simulink model "winder_mechanics"  (R2026a)
settings: Solver=VariableStepAuto  StopTime=Tsim  MaxStep=1e-3  RelTol=1e-4
undefined symbols (not defined in the file): draw_max, F_ref, Ki_draw, Ki_speed, Kp_draw, Kp_speed, Tmax, v_init, v_max, v_slope, winder_mode
libraries: slpidlib x2, simulink x1
settings Model: Creator=kunal  LastModifiedBy=kunal

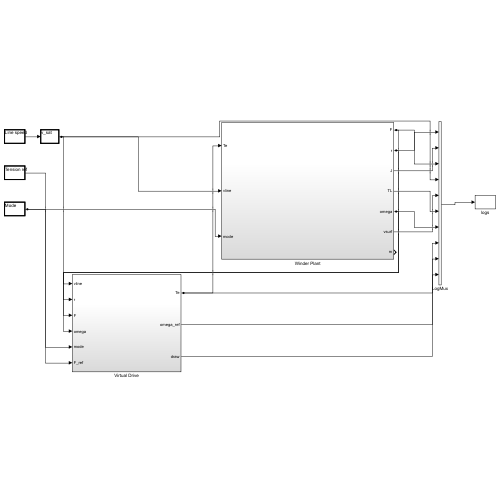
[thumbnail: Simulink's stored preview of the top-level diagram]
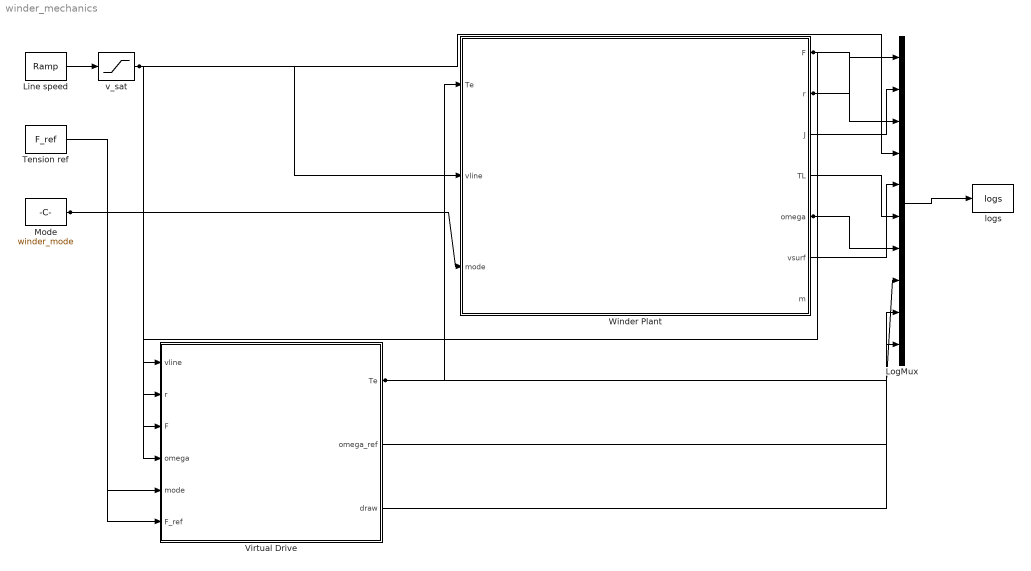
== system winder_mechanics ==
  Line speed : simulink/Sources/Ramp  slope=v_slope  start=0  InitialOutput=v_init
  LogMux : Mux  Inputs=10
  Mode : Constant  Value=winder_mode
  Tension ref : Constant  Value=F_ref
  Virtual Drive : Subsystem
  Winder Plant : Subsystem
  logs : ToWorkspace  VariableName=logs  SaveFormat=Timeseries  SampleTime=-1
  v_sat : Saturate  UpperLimit=v_max  LowerLimit=0
  wires:
  Line speed/1 -> v_sat/1
  v_sat/1 -> Winder Plant/2(vline), Virtual Drive/1(vline), LogMux/4
  Tension ref/1 -> Virtual Drive/6(F_ref)
  Mode/1 -> Winder Plant/3(mode), Virtual Drive/5(mode)
  Winder Plant/2(r) -> Virtual Drive/2(r), LogMux/1
  Winder Plant/1(F) -> Virtual Drive/3(F), LogMux/3
  Winder Plant/5(omega) -> Virtual Drive/4(omega), LogMux/7
  Virtual Drive/1(Te) -> Winder Plant/1(Te), LogMux/8
  Winder Plant/3(J) -> LogMux/2
  Winder Plant/6(vsurf) -> LogMux/5
  Winder Plant/4(TL) -> LogMux/6
  Virtual Drive/2(omega_ref) -> LogMux/9
  Virtual Drive/3(draw) -> LogMux/10
  LogMux/1 -> logs/1

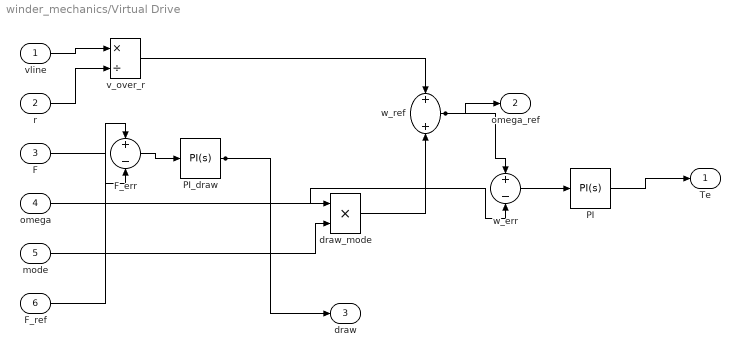
== system winder_mechanics/Virtual Drive ==
  vline : Inport
  r : Inport  Port=2
  F : Inport  Port=3
  omega : Inport  Port=4
  mode : Inport  Port=5
  F_ref : Inport  Port=6
  F_err : Sum  Inputs=+-
  PI : slpidlib/PID Controller  Controller=PI  Form=Parallel  TimeDomain=Continuous-time  UseExternalTs=off  SampleTime=-1  IntegratorMethod=Forward Euler  FilterMethod=Forward Euler  ControllerParametersSource=internal  P=Kp_speed  I=Ki_speed  UseKiTs=off  D=0  UseExternalDerivativeSource=off  N=100  UseFilter=on  TunerSelectOption=Transfer Function Based (PID Tuner App)  InitialConditionSource=internal  InitialConditionForIntegrator=Te0  InitialConditionForFilter=0  DifferentiatorICPrevScaledInput=0  ExternalReset=none  TrackingMode=off  Kt=1  LimitOutput=on  SatLimitsSource=internal  UpperSaturationLimit=Tmax  LowerSaturationLimit=-Tmax  LinearizeAsGain=on  AntiWindupMode=clamping  Kb=1  LimitIntegrator=off  UpperIntegratorSaturationLimit=inf  LowerIntegratorSaturationLimit=-inf  POutMin=[]  POutMax=[]  IOutMin=[]  IOutMax=[]  DOutMin=[]  DOutMax=[]  NOutMin=[]  NOutMax=[]  SumOutMin=[]  SumOutMax=[]  SaturationOutMin=[]  SaturationOutMax=[]  PParamMin=[]  PParamMax=[]  IParamMin=[]  IParamMax=[]  DParamMin=[]  DParamMax=[]  NParamMin=[]  NParamMax=[]  KbParamMin=[]  KbParamMax=[]  KtParamMin=[]  KtParamMax=[]  KbOutMin=[]  KbOutMax=[]  KtOutMin=[]  KtOutMax=[]  IntegratorOutMin=[]  IntegratorOutMax=[]  FilterOutMin=[]  FilterOutMax=[]  SumI1OutMin=[]  SumI1OutMax=[]  SumI2OutMin=[]  SumI2OutMax=[]  SumI3OutMin=[]  SumI3OutMax=[]  SumI4OutMin=[]  SumI4OutMax=[]  SumDOutMin=[]  SumDOutMax=[]  DifferentiatorOutMin=[]  DifferentiatorOutMax=[]  FilterDiffOutCoefMin=[]  FilterDiffOutCoefMax=[]  ReciprocalOutMin=[]  ReciprocalOutMax=[]  SumDenOutMin=[]  SumDenOutMax=[]  SumNumOutMin=[]  SumNumOutMax=[]  DivideOutMin=[]  DivideOutMax=[]  UdiffTsProdOutMin=[]  UdiffTsProdOutMax=[]  NTsProdOutMin=[]  NTsProdOutMax=[]  UintegralTsProdOutMin=[]  UintegralTsProdOutMax=[]  UngainTsProdOutMin=[]  UngainTsProdOutMax=[]  ClampingZeroOutDataTypeStr=Inherit: Inherit via back propagation  ClampingZeroOutMin=[]  ClampingZeroOutMax=[]  FilterDenConstantOutDataTypeStr=Inherit: Inherit via back propagation  FilterDenConstantOutMin=[]  FilterDenConstantOutMax=[]  PCopyOutDataTypeStr=Inherit: Inherit via back propagation  PCopyOutMin=[]  PCopyOutMax=[]  NCopyOutDataTypeStr=Inherit: Inherit via back propagation  NCopyOutMin=[]  NCopyOutMax=[]  IntegratorContinuousStateAttributes=''  IntegratorStateMustResolveToSignalObject=off  IntegratorRTWStateStorageClass=Auto  FilterContinuousStateAttributes=''  FilterStateMustResolveToSignalObject=off  FilterRTWStateStorageClass=Auto  ParallelPVariant=InternalParameters  IdealPVariant=Disabled  IVariant=InternalParameters  DVariant=Disabled  IntegratorVariant=Continuous  SatVariant=Enabled  AWVariant=ContClampingParallel  PCopyVariant=Disabled  TRVariant=Disabled  FdbkBlocksVariant=Forward  IdealPFdbkVariant=Disabled  SatFdbkVariant=Disabled  DerivativeFilterVariant=Disabled  NVariant=Disabled  NCopyVariant=Disabled_SignalSpec  FilterICVariant=Disabled  IntegratorICVariant=InternalICs  ExternalResetVariant=Disabled  TRSumVariant=Passthrough  SumFdbkVariant=Disabled  SumVariant=Sum_PI  TsampFilterVariant=InternalTs  TsampNgainVariant=Passthrough  TsampIntegralVariant=Disabled_SignalSpec  ExternalSaturationOutDataTypeStr=Inherit: Same as second input  DerivativeSourceVariant=Disabled  PreIntVariant=InternalPreInt
  PI_draw : slpidlib/PID Controller  Controller=PI  Form=Parallel  TimeDomain=Continuous-time  UseExternalTs=off  SampleTime=-1  IntegratorMethod=Forward Euler  FilterMethod=Forward Euler  ControllerParametersSource=internal  P=Kp_draw  I=Ki_draw  UseKiTs=off  D=0  UseExternalDerivativeSource=off  N=100  UseFilter=on  TunerSelectOption=Transfer Function Based (PID Tuner App)  InitialConditionSource=internal  InitialConditionForIntegrator=0  InitialConditionForFilter=0  DifferentiatorICPrevScaledInput=0  ExternalReset=none  TrackingMode=off  Kt=1  LimitOutput=on  SatLimitsSource=internal  UpperSaturationLimit=draw_max  LowerSaturationLimit=-draw_max  LinearizeAsGain=on  AntiWindupMode=clamping  Kb=1  LimitIntegrator=off  UpperIntegratorSaturationLimit=inf  LowerIntegratorSaturationLimit=-inf  POutMin=[]  POutMax=[]  IOutMin=[]  IOutMax=[]  DOutMin=[]  DOutMax=[]  NOutMin=[]  NOutMax=[]  SumOutMin=[]  SumOutMax=[]  SaturationOutMin=[]  SaturationOutMax=[]  PParamMin=[]  PParamMax=[]  IParamMin=[]  IParamMax=[]  DParamMin=[]  DParamMax=[]  NParamMin=[]  NParamMax=[]  KbParamMin=[]  KbParamMax=[]  KtParamMin=[]  KtParamMax=[]  KbOutMin=[]  KbOutMax=[]  KtOutMin=[]  KtOutMax=[]  IntegratorOutMin=[]  IntegratorOutMax=[]  FilterOutMin=[]  FilterOutMax=[]  SumI1OutMin=[]  SumI1OutMax=[]  SumI2OutMin=[]  SumI2OutMax=[]  SumI3OutMin=[]  SumI3OutMax=[]  SumI4OutMin=[]  SumI4OutMax=[]  SumDOutMin=[]  SumDOutMax=[]  DifferentiatorOutMin=[]  DifferentiatorOutMax=[]  FilterDiffOutCoefMin=[]  FilterDiffOutCoefMax=[]  ReciprocalOutMin=[]  ReciprocalOutMax=[]  SumDenOutMin=[]  SumDenOutMax=[]  SumNumOutMin=[]  SumNumOutMax=[]  DivideOutMin=[]  DivideOutMax=[]  UdiffTsProdOutMin=[]  UdiffTsProdOutMax=[]  NTsProdOutMin=[]  NTsProdOutMax=[]  UintegralTsProdOutMin=[]  UintegralTsProdOutMax=[]  UngainTsProdOutMin=[]  UngainTsProdOutMax=[]  ClampingZeroOutDataTypeStr=Inherit: Inherit via back propagation  ClampingZeroOutMin=[]  ClampingZeroOutMax=[]  FilterDenConstantOutDataTypeStr=Inherit: Inherit via back propagation  FilterDenConstantOutMin=[]  FilterDenConstantOutMax=[]  PCopyOutDataTypeStr=Inherit: Inherit via back propagation  PCopyOutMin=[]  PCopyOutMax=[]  NCopyOutDataTypeStr=Inherit: Inherit via back propagation  NCopyOutMin=[]  NCopyOutMax=[]  IntegratorContinuousStateAttributes=''  IntegratorStateMustResolveToSignalObject=off  IntegratorRTWStateStorageClass=Auto  FilterContinuousStateAttributes=''  FilterStateMustResolveToSignalObject=off  FilterRTWStateStorageClass=Auto  ParallelPVariant=InternalParameters  IdealPVariant=Disabled  IVariant=InternalParameters  DVariant=Disabled  IntegratorVariant=Continuous  SatVariant=Enabled  AWVariant=ContClampingParallel  PCopyVariant=Disabled  TRVariant=Disabled  FdbkBlocksVariant=Forward  IdealPFdbkVariant=Disabled  SatFdbkVariant=Disabled  DerivativeFilterVariant=Disabled  NVariant=Disabled  NCopyVariant=Disabled_SignalSpec  FilterICVariant=Disabled  IntegratorICVariant=InternalICs  ExternalResetVariant=Disabled  TRSumVariant=Passthrough  SumFdbkVariant=Disabled  SumVariant=Sum_PI  TsampFilterVariant=InternalTs  TsampNgainVariant=Passthrough  TsampIntegralVariant=Disabled_SignalSpec  ExternalSaturationOutDataTypeStr=Inherit: Same as second input  DerivativeSourceVariant=Disabled  PreIntVariant=InternalPreInt
  draw_mode : Product
  v_over_r : Product  Inputs=*/
  w_err : Sum  Inputs=+-
  w_ref : Sum
  Te : Outport
  omega_ref : Outport  Port=2
  draw : Outport  Port=3
  wires:
  vline/1 -> v_over_r/1
  r/1 -> v_over_r/2
  F_ref/1 -> F_err/1
  F/1 -> F_err/2
  F_err/1 -> PI_draw/1
  PI_draw/1 -> draw_mode/1, draw/1
  mode/1 -> draw_mode/2
  v_over_r/1 -> w_ref/1
  draw_mode/1 -> w_ref/2
  w_ref/1 -> w_err/1, omega_ref/1
  omega/1 -> w_err/2
  w_err/1 -> PI/1
  PI/1 -> Te/1

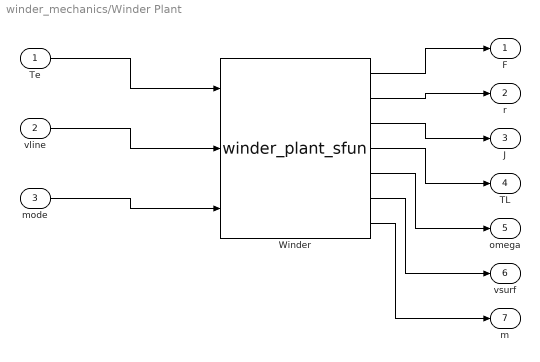
== system winder_mechanics/Winder Plant ==
  Te : Inport
  vline : Inport  Port=2
  mode : Inport  Port=3
  Winder : M-S-Function  FunctionName=winder_plant_sfun  Parameters=winder_p, r0, H0, F0
  F : Outport
  r : Outport  Port=2
  J : Outport  Port=3
  TL : Outport  Port=4
  omega : Outport  Port=5
  vsurf : Outport  Port=6
  m : Outport  Port=7
  wires:
  Te/1 -> Winder/1
  vline/1 -> Winder/2
  mode/1 -> Winder/3
  Winder/1 -> F/1
  Winder/2 -> r/1
  Winder/3 -> J/1
  Winder/4 -> TL/1
  Winder/5 -> omega/1
  Winder/6 -> vsurf/1
  Winder/7 -> m/1
